simulink model "SimuHInf"  (R2023b)
settings: Solver=VariableStepAuto  StartTime=0.0  StopTime=100  RelTol=1e-3
values from neighbouring files (symbols this model uses):
  SysLong = ss(Along,Blong,Clong,Dlong)    [PIDComplelto.m]    (also in T1_Hinf_Dir.m = ss(Anew,Bnew,Cnew,Dnew); T1_Hinf_Dir_v2.m = ss(Anew,Bnew,Cnew,Dnew); T1_Hinf_Lat.m = ss(Anew,Bnew,Cnew,Dnew); T1_Hinf_Long.m = ss(Anew,Bnew,Cnew,Dnew))
undefined symbols (not defined in the file or in its folder): K1
libraries: simulink x1
settings Model: Creator=sslan  LastModifiedBy=sslan

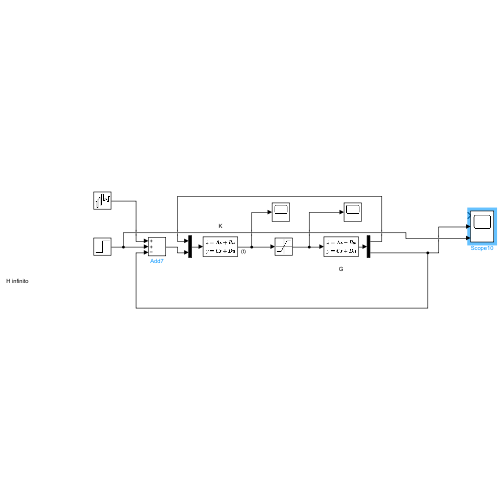
[thumbnail: Simulink's stored preview of the top-level diagram]
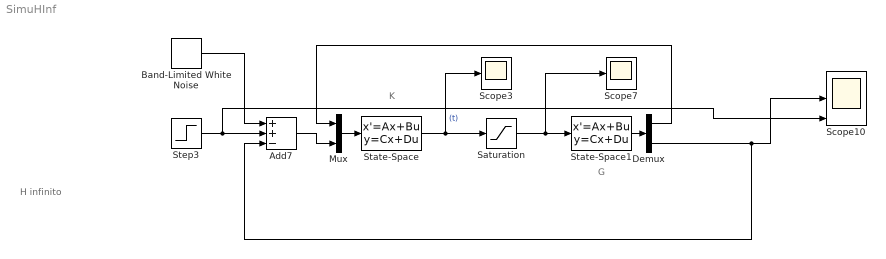
== system SimuHInf ==
  note: G
  note: H infinito
  note: K
  Add7 : Sum  Inputs=++-
  Band-Limited White Noise : simulink/Sources/Band-Limited White Noise  Cov=[0.001]  Ts=0.01  seed=[23341]
  Demux : Demux  Outputs=2
  Mux : Mux  Inputs=2
  Saturation : Saturate  UpperLimit=30  LowerLimit=-30
  Scope10 : Scope  NumInputPorts=3
  Scope3 : Scope
  Scope7 : Scope
  State-Space : StateSpace  A=K1.A  B=K1.B  C=K1.C  D=K1.D  InitialCondition=0
  State-Space1 : StateSpace  A=SysLong.A  B=SysLong.B  C=SysLong.C  D=SysLong.D  InitialCondition=0
  Step3 : Step  Time=15  Before=-40  After=40  SampleTime=0
  wires:
  State-Space/1 -> Saturation/1, Scope3/1  "(t)"
  Saturation/1 -> State-Space1/1, Scope7/1
  Step3/1 -> Scope10/3, Add7/2
  Mux/1 -> State-Space/1
  State-Space1/1 -> Demux/1
  Demux/1 -> Mux/1
  Add7/1 -> Mux/2
  Demux/2 -> Add7/3, Scope10/2
  Band-Limited White Noise/1 -> Add7/1
